simulink model "MATLAB_Arduino_ICM42688P"  (R2021a)
settings: Solver=VariableStepAuto  StartTime=0.0  StopTime=10.0  RelTol=1e-3
libraries: arduinolib x9
settings Model: Creator=mpnoy  LastModifiedBy=mpnoy

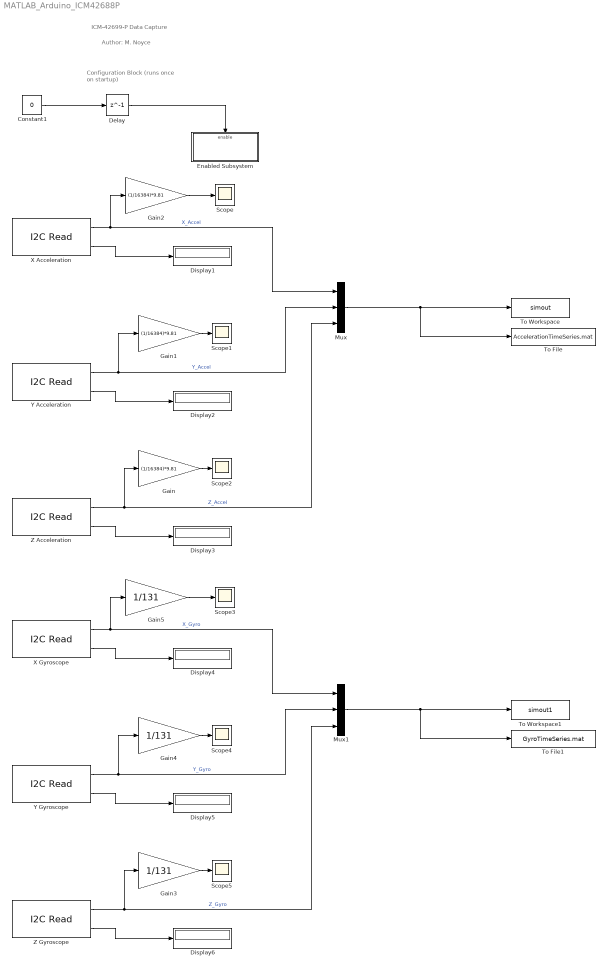
== system MATLAB_Arduino_ICM42688P ==
  note: Configuration Block
      | (runs once on startup)
  note: ICM-42699-P Data Capture
  note: Author: M. Noyce
  Constant1 : Constant  Value=0
  Delay : Delay  DelayLength=1  InitialCondition=1
  Display{1..6} (6 alike) : Display
  Enabled Subsystem : Subsystem  TreatAsAtomicUnit=on
  Gain : Gain  Gain=(1/16384)*9.81
  Gain1 : Gain  Gain=(1/16384)*9.81
  Gain2 : Gain  Gain=(1/16384)*9.81
  Gain3 : Gain  Gain=1/131
  Gain4 : Gain  Gain=1/131
  Gain5 : Gain  Gain=1/131
  Mux : Mux  Inputs=3
  Mux1 : Mux  Inputs=3
  Scope{,1..5} (6 alike) : Scope
  To File : ToFile  Filename=AccelerationTimeSeries.mat  MatrixName=Acceleration  SaveFormat=Timeseries
  To File1 : ToFile  Filename=GyroTimeSeries.mat  MatrixName=Orientation  SaveFormat=Timeseries
  To Workspace : ToWorkspace  VariableName=simout  SaveFormat=Timeseries  SampleTime=-1
  To Workspace1 : ToWorkspace  VariableName=simout1  SaveFormat=Timeseries  SampleTime=-1
  "X Acceleration " : arduinolib/I2C Read  I2CModule=0  Mode=Master  SlaveAddress=104  SlaveByteOrder=BigEndian  Direction=Receiver  RegisterAddressMode=on  RegisterAddress=uint8(hex2dec('1F'))  SlaveDataType=int16  DataLength=1  NoAck=off  RepeatedStart=off  OutputStatus=on  blockPlatform=ARDUINO  SampleTime=0.01
      settings: SourceProductBaseCode=ARDUINO
  X Gyroscope : arduinolib/I2C Read  I2CModule=0  Mode=Master  SlaveAddress=104  SlaveByteOrder=BigEndian  Direction=Receiver  RegisterAddressMode=on  RegisterAddress=uint8(hex2dec('43'))  SlaveDataType=int16  DataLength=1  NoAck=off  RepeatedStart=off  OutputStatus=on  blockPlatform=ARDUINO  SampleTime=0.01
      settings: SourceProductBaseCode=ARDUINO
  Y Acceleration : arduinolib/I2C Read  I2CModule=0  Mode=Master  SlaveAddress=104  SlaveByteOrder=BigEndian  Direction=Receiver  RegisterAddressMode=on  RegisterAddress=uint8(hex2dec('22'))  SlaveDataType=int16  DataLength=1  NoAck=off  RepeatedStart=off  OutputStatus=on  blockPlatform=ARDUINO  SampleTime=0.01
      settings: SourceProductBaseCode=ARDUINO
  Y Gyroscope : arduinolib/I2C Read  I2CModule=0  Mode=Master  SlaveAddress=104  SlaveByteOrder=BigEndian  Direction=Receiver  RegisterAddressMode=on  RegisterAddress=uint8(hex2dec('45'))  SlaveDataType=int16  DataLength=1  NoAck=off  RepeatedStart=off  OutputStatus=on  blockPlatform=ARDUINO  SampleTime=0.01
      settings: SourceProductBaseCode=ARDUINO
  "Z Acceleration " : arduinolib/I2C Read  I2CModule=0  Mode=Master  SlaveAddress=104  SlaveByteOrder=BigEndian  Direction=Receiver  RegisterAddressMode=on  RegisterAddress=uint8(hex2dec('3F'))  SlaveDataType=int16  DataLength=1  NoAck=off  RepeatedStart=off  OutputStatus=on  blockPlatform=ARDUINO  SampleTime=0.01
      settings: SourceProductBaseCode=ARDUINO
  Z Gyroscope : arduinolib/I2C Read  I2CModule=0  Mode=Master  SlaveAddress=104  SlaveByteOrder=BigEndian  Direction=Receiver  RegisterAddressMode=on  RegisterAddress=uint8(hex2dec('47'))  SlaveDataType=int16  DataLength=1  NoAck=off  RepeatedStart=off  OutputStatus=on  blockPlatform=ARDUINO  SampleTime=0.01
      settings: SourceProductBaseCode=ARDUINO
  wires:
  "X Acceleration "/1 -> Mux/1, Gain2/1  "X_Accel"
  "X Acceleration "/2 -> Display1/1
  Constant1/1 -> Delay/1
  Z Gyroscope/1 -> Mux1/3, Gain3/1  "Z_Gyro"
  Z Gyroscope/2 -> Display6/1
  Y Gyroscope/1 -> Mux1/2, Gain4/1  "Y_Gyro"
  Mux1/1 -> To File1/1, To Workspace1/1
  Mux/1 -> To File/1, To Workspace/1
  Gain/1 -> Scope2/1
  Y Acceleration/2 -> Display2/1
  Gain3/1 -> Scope5/1
  Y Gyroscope/2 -> Display5/1
  Gain1/1 -> Scope1/1
  X Gyroscope/1 -> Mux1/1, Gain5/1  "X_Gyro"
  "Z Acceleration "/2 -> Display3/1
  Gain2/1 -> Scope/1
  Gain4/1 -> Scope4/1
  Delay/1 -> Enabled Subsystem/Enable
  Y Acceleration/1 -> Mux/2, Gain1/1  "Y_Accel"
  "Z Acceleration "/1 -> Mux/3, Gain/1  "Z_Accel"
  Gain5/1 -> Scope3/1
  X Gyroscope/2 -> Display4/1

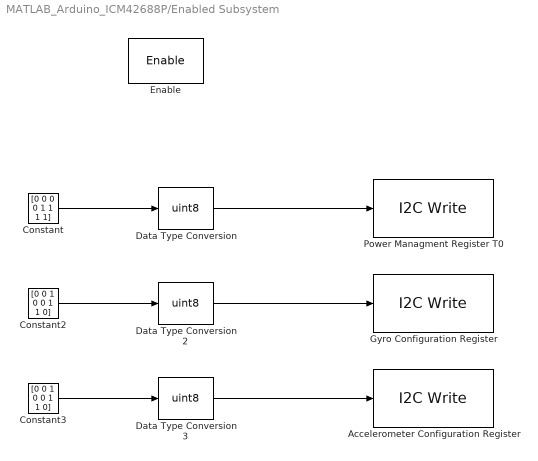
== system MATLAB_Arduino_ICM42688P/Enabled Subsystem ==
  Enable : EnablePort
  "Accelerometer Configuration Register " : arduinolib/I2C Write  I2CModule=0  Mode=Master  SlaveAddress=104  SlaveByteOrder=BigEndian  Direction=Transmitter  RegisterAddressMode=on  RegisterAddress=uint8(hex2dec('1C'))  SlaveDataType=uint8  DataLength=1  NoAck=off  RepeatedStart=off  OutputStatus=off  blockPlatform=ARDUINO
      settings: SourceProductBaseCode=ARDUINO
  Constant : Constant  Value=[0 0 0 0 1 1 1 1]
  Constant2 : Constant  Value=[0 0 1 0 0 1 1 0]
  Constant3 : Constant  Value=[0 0 1 0 0 1 1 0]
  Data Type Conversion : DataTypeConversion  OutDataTypeStr=uint8
  Data Type Conversion2 : DataTypeConversion  OutDataTypeStr=uint8
  Data Type Conversion3 : DataTypeConversion  OutDataTypeStr=uint8
  Gyro Configuration Register : arduinolib/I2C Write  I2CModule=0  Mode=Master  SlaveAddress=104  SlaveByteOrder=BigEndian  Direction=Transmitter  RegisterAddressMode=on  RegisterAddress=uint8(hex2dec('4F'))  SlaveDataType=uint8  DataLength=1  NoAck=off  RepeatedStart=off  OutputStatus=off  blockPlatform=ARDUINO
      settings: SourceProductBaseCode=ARDUINO
  "Power Managment Register T0 " : arduinolib/I2C Write  I2CModule=0  Mode=Master  SlaveAddress=104  SlaveByteOrder=BigEndian  Direction=Transmitter  RegisterAddressMode=on  RegisterAddress=uint8(hex2dec('6B'))  SlaveDataType=uint8  DataLength=1  NoAck=off  RepeatedStart=off  OutputStatus=off  blockPlatform=ARDUINO
      settings: SourceProductBaseCode=ARDUINO
  wires:
  Data Type Conversion/1 -> "Power Managment Register T0 "/1
  Constant/1 -> Data Type Conversion/1
  Data Type Conversion2/1 -> Gyro Configuration Register/1
  Constant2/1 -> Data Type Conversion2/1
  Data Type Conversion3/1 -> "Accelerometer Configuration Register "/1
  Constant3/1 -> Data Type Conversion3/1
